simulink model "AFC2_F_trainscg_15_15_15_15_controller_ep_500_Nor_20250717"  (R2021a)
settings: Solver=VariableStepAuto  StartTime=0.0  StopTime=10.0  RelTol=1e-3
libraries: neural x66
(part 2 of 3)

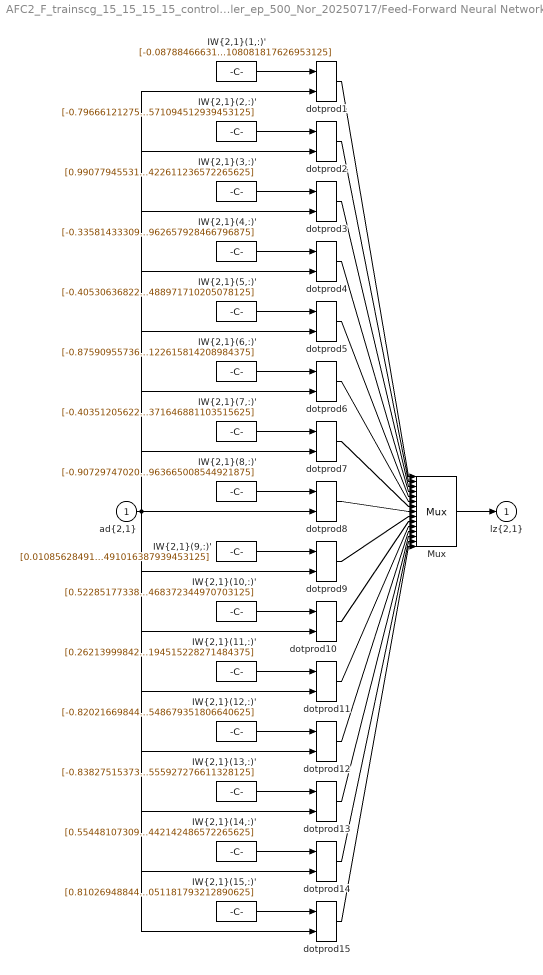
== system AFC2_F_trainscg_15_15_15_15_controller_ep_500_Nor_20250717/Feed-Forward Neural Network/Layer 2/LW{2,1} ==
  "ad{2,1}" : Inport  PortDimensions=15
      mask Display: e = 0.06;c1 = [120 230 180]/255;c2 = ([120 230 180]+0)/(256+128);c3 = ([120 230 180]+128)/(256+128);patch([0 1 1 0],[0 0 1 1],c1);patch([0 1 1 1-e 1-e 0+e],[0 0 1 1-e 0+e 0+e],c2);patch([0 0 1 1-e 0+e 0+e],[0 1 1 1-e 1-e 0+e],c3);plot([0 1 1 0 0],[0 0 1 1 0]);
  "IW{2,1}(1,:)'" : Constant  Value=[-0.0878846663125170124430951545946300029754638671875;0.06775174892635017764863647471429430879652500152587890625;0.385060464315723993689033477494376711547374725341796875;-0.8973191118577101832443077000789344310760498046875;0.4800646559755552544856982422061264514923095703125;-0.60641376213614639478777235126472078263759613037109375;-0.7754320756879466980393544872640632092952728271484375;-0.03645452907563362376919258167617954313755035400390625;-0.81526323382648147042317532395827583968639373779296875;-0.367884988017231240320370488916523754596710205078125;0.97615990087424953092209989335970021784305572509765625;-0.31661933240200113015561100837658159434795379638671875;-0.7502406969507842138256137332064099609851837158203125;-0.07347884281256167327001094236038625240325927734375;0.61840770258758670507859278586693108081817626953125]
      mask Display: e = 0.06;c1 = [120 150 230]/255;c2 = ([120 150 230]+0)/383;c3 = ([120 150 230]+128)/383;patch([0 1 1 0],[0 0 1 1],c1);patch([0 1 1 1-e 1-e 0+e],[0 0 1 1-e 0+e 0+e],c2);patch([0 0 1 1-e 0+e 0+e],[0 1 1 1-e 1-e 0+e],c3);plot([0 1 1 0 0],[0 0 1 1 0]);disp('weights');
  "IW{2,1}(10,:)'" : Constant  Value=[0.5228517733802267031251176376827061176300048828125;0.20693596766153898869333715992979705333709716796875;-0.7442232404340096696415685073588974773883819580078125;-0.7650142956963341678289225455955602228641510009765625;0.1958832707677782281052714097313582897186279296875;-0.4115421196069359854874392112833447754383087158203125;0.3109960796070747601760331235709600150585174560546875;-0.88112125053411405328773753353743813931941986083984375;-0.731393391372850754095225056516937911510467529296875;0.82788407804859354133242277384852059185504913330078125;0.2413438943991568219615828638779930770397186279296875;-0.154255850726072007983447065271320752799510955810546875;0.5277958885729565619016057098633609712123870849609375;0.4054046139009506166672736071632243692874908447265625;-0.489226519023898465121646950137801468372344970703125]
      mask Display: e = 0.06;c1 = [120 150 230]/255;c2 = ([120 150 230]+0)/383;c3 = ([120 150 230]+128)/383;patch([0 1 1 0],[0 0 1 1],c1);patch([0 1 1 1-e 1-e 0+e],[0 0 1 1-e 0+e 0+e],c2);patch([0 0 1 1-e 0+e 0+e],[0 1 1 1-e 1-e 0+e],c3);plot([0 1 1 0 0],[0 0 1 1 0]);disp('weights');
  "IW{2,1}(11,:)'" : Constant  Value=[0.262139998427187048690711890230886638164520263671875;0.0522049315911223832387122456566430628299713134765625;0.0990802140303959077982653980143368244171142578125;0.2814358459318511140878626974881626665592193603515625;0.5787278872838108600973328066174872219562530517578125;-0.5252539605888415508161415345966815948486328125;-0.780489898553896832567033925442956387996673583984375;-0.3683771233222679075680616733734495937824249267578125;-0.8028118145780045455950357791152782738208770751953125;0.4134304353938611509278189259930513799190521240234375;-0.691260389041455258762880475842393934726715087890625;-0.2807873640555287320097477277158759534358978271484375;0.518654766262192534753694417304359376430511474609375;-0.692819246761199547535170495393685996532440185546875;-0.9589284506836308619170949896215461194515228271484375]
      mask Display: e = 0.06;c1 = [120 150 230]/255;c2 = ([120 150 230]+0)/383;c3 = ([120 150 230]+128)/383;patch([0 1 1 0],[0 0 1 1],c1);patch([0 1 1 1-e 1-e 0+e],[0 0 1 1-e 0+e 0+e],c2);patch([0 0 1 1-e 0+e 0+e],[0 1 1 1-e 1-e 0+e],c3);plot([0 1 1 0 0],[0 0 1 1 0]);disp('weights');
  "IW{2,1}(12,:)'" : Constant  Value=[-0.8202166984478165279170980284106917679309844970703125;0.2472596760229174017720055189784034155309200286865234375;-0.03130315437321791460778541704712552018463611602783203125;-0.25779005620817307953274166720802895724773406982421875;-0.26469416312424609571962719201110303401947021484375;0.273188766533149329784890824157628230750560760498046875;0.86751969677066487207639511325396597385406494140625;0.6303759335450056511263028369285166263580322265625;-0.69044021123110133064670890234992839395999908447265625;-0.023850347134512041302745188886547111906111240386962890625;-0.211816580907498830388391297674388624727725982666015625;0.06174872535074608925764749756126548163592815399169921875;0.481829751237097259064512400072999298572540283203125;0.90691413977249535349756115465424954891204833984375;0.8473512252408144096449404969462193548679351806640625]
      mask Display: e = 0.06;c1 = [120 150 230]/255;c2 = ([120 150 230]+0)/383;c3 = ([120 150 230]+128)/383;patch([0 1 1 0],[0 0 1 1],c1);patch([0 1 1 1-e 1-e 0+e],[0 0 1 1-e 0+e 0+e],c2);patch([0 0 1 1-e 0+e 0+e],[0 1 1 1-e 1-e 0+e],c3);plot([0 1 1 0 0],[0 0 1 1 0]);disp('weights');
  "IW{2,1}(13,:)'" : Constant  Value=[-0.8382751537393726692926065879873931407928466796875;0.414506970630843074587801311281509697437286376953125;0.7809513583688765248069785229745320975780487060546875;0.3076240451915472906563309152261354029178619384765625;-0.5879442809896107124956188272335566580295562744140625;-0.82060262315297738400232674393919296562671661376953125;-0.62507838715662700224129366688430309295654296875;0.38755084301493669673988051727064885199069976806640625;-0.6634974030169444869642347839544527232646942138671875;-0.374899537179466724179377479231334291398525238037109375;-0.6777314823067481786011967415106482803821563720703125;0.47876521781964653801111353459418751299381256103515625;0.4873766829746519757549094720161519944667816162109375;0.0817681624829529329900879019987769424915313720703125;0.3073997780165058646417719501187093555927276611328125]
      mask Display: e = 0.06;c1 = [120 150 230]/255;c2 = ([120 150 230]+0)/383;c3 = ([120 150 230]+128)/383;patch([0 1 1 0],[0 0 1 1],c1);patch([0 1 1 1-e 1-e 0+e],[0 0 1 1-e 0+e 0+e],c2);patch([0 0 1 1-e 0+e 0+e],[0 1 1 1-e 1-e 0+e],c3);plot([0 1 1 0 0],[0 0 1 1 0]);disp('weights');
  "IW{2,1}(14,:)'" : Constant  Value=[0.554481073097886412170964831602759659290313720703125;0.5627541035985543782516060673515312373638153076171875;0.597920557625758686270955877262167632579803466796875;0.498262926207038159276407895958982408046722412109375;-0.8266669052089354874368609671364538371562957763671875;-0.189369160238817446639814079389907419681549072265625;-0.4676423221847223476999033664469607174396514892578125;-0.7493356377816400293312426583725027740001678466796875;-0.6075021554860893235883168017608113586902618408203125;-0.6675928741956986822714270601863972842693328857421875;0.516224862654837135522711832891218364238739013671875;-0.1513304327486186817708357921219430863857269287109375;-0.7881591665344693797834452198003418743610382080078125;0.3594677964209338494327994339982978999614715576171875;0.8652271440971281979415152818546630442142486572265625]
      mask Display: e = 0.06;c1 = [120 150 230]/255;c2 = ([120 150 230]+0)/383;c3 = ([120 150 230]+128)/383;patch([0 1 1 0],[0 0 1 1],c1);patch([0 1 1 1-e 1-e 0+e],[0 0 1 1-e 0+e 0+e],c2);patch([0 0 1 1-e 0+e 0+e],[0 1 1 1-e 1-e 0+e],c3);plot([0 1 1 0 0],[0 0 1 1 0]);disp('weights');
  "IW{2,1}(15,:)'" : Constant  Value=[0.810269488447141750242508351220749318599700927734375;-0.424046048771657524412148632109165191650390625;0.4686821673919394637408686321577988564968109130859375;0.1663714629097523545198100691777653992176055908203125;0.543867834198214605834209578461013734340667724609375;-0.790307304190327020165796056971885263919830322265625;0.5956605204231941730341759466682560741901397705078125;-0.7396970992211528983517609958653338253498077392578125;-0.36504044970112925483363142120651900768280029296875;0.244994582064439025970159491407684981822967529296875;0.7422222438307783942690321055124513804912567138671875;-0.1412881308849082417911091624773689545691013336181640625;0.3631208609406313403411559193045832216739654541015625;-0.926873963903094288951933776843361556529998779296875;-0.6729752629449488043889004984521307051181793212890625]
      mask Display: e = 0.06;c1 = [120 150 230]/255;c2 = ([120 150 230]+0)/383;c3 = ([120 150 230]+128)/383;patch([0 1 1 0],[0 0 1 1],c1);patch([0 1 1 1-e 1-e 0+e],[0 0 1 1-e 0+e 0+e],c2);patch([0 0 1 1-e 0+e 0+e],[0 1 1 1-e 1-e 0+e],c3);plot([0 1 1 0 0],[0 0 1 1 0]);disp('weights');
  "IW{2,1}(2,:)'" : Constant  Value=[-0.7966612127504897333807321047061122953891754150390625;-1.0766944439080428086441543200635351240634918212890625;0.1082001892355971273129711107685579918324947357177734375;-0.7153346012591350611131701953127048909664154052734375;-0.530346170504191416483763532596640288829803466796875;-0.112530674013214093687196282189688645303249359130859375;0.5688557814878254514923128226655535399913787841796875;0.65169344071455370670520323983510024845600128173828125;-0.9528829808403223022850170309538953006267547607421875;-0.498930486024516006704487836032058112323284149169921875;-0.64958838734927548674846775611513294279575347900390625;0.35345638821586522482220971141941845417022705078125;-0.94870227449216282256116983262472786009311676025390625;-0.5756735894901312544646998503594659268856048583984375;0.4972377435523942512674011595663614571094512939453125]
      mask Display: e = 0.06;c1 = [120 150 230]/255;c2 = ([120 150 230]+0)/383;c3 = ([120 150 230]+128)/383;patch([0 1 1 0],[0 0 1 1],c1);patch([0 1 1 1-e 1-e 0+e],[0 0 1 1-e 0+e 0+e],c2);patch([0 0 1 1-e 0+e 0+e],[0 1 1 1-e 1-e 0+e],c3);plot([0 1 1 0 0],[0 0 1 1 0]);disp('weights');
  "IW{2,1}(3,:)'" : Constant  Value=[0.9907794553101834100772293822956271469593048095703125;0.64699276355253754200447247058036737143993377685546875;-0.20695841483681487460444259340874850749969482421875;-0.82294508093848228735822658563847653567790985107421875;0.4699150833921044156937796287820674479007720947265625;0.06427580211802334797521751852400484494864940643310546875;-0.416859364186138225960576164652593433856964111328125;-0.2080844447464574031858575153819401748478412628173828125;-0.15378122955226392054584039215114898979663848876953125;-0.497960891694102125715204465450369752943515777587890625;-0.4844154988559739027920159060158766806125640869140625;-0.438200669103228801493088440111023373901844024658203125;-0.419629630291659949659077710748533718287944793701171875;-0.8029625246237832580931126358336769044399261474609375;-0.7596259640258387069167156369076110422611236572265625]
      mask Display: e = 0.06;c1 = [120 150 230]/255;c2 = ([120 150 230]+0)/383;c3 = ([120 150 230]+128)/383;patch([0 1 1 0],[0 0 1 1],c1);patch([0 1 1 1-e 1-e 0+e],[0 0 1 1-e 0+e 0+e],c2);patch([0 0 1 1-e 0+e 0+e],[0 1 1 1-e 1-e 0+e],c3);plot([0 1 1 0 0],[0 0 1 1 0]);disp('weights');
  "IW{2,1}(4,:)'" : Constant  Value=[-0.335814333095001860129968918045051395893096923828125;-0.3238045623956562479861531755886971950531005859375;-0.8768186658920706921804821831756271421909332275390625;0.5967017282279047929449689036118797957897186279296875;0.94119705017322896622999905957840383052825927734375;-0.54119677378130448541782016036449931561946868896484375;0.207066877501773660696926526725292205810546875;-0.453886991560920105559517878646147437393665313720703125;0.3111463498758286760903501999564468860626220703125;0.786704430823791600602135076769627630710601806640625;-0.2064013627337126788319210390909574925899505615234375;0.06251065725207975709576402323364163748919963836669921875;-0.3649588342015472886004090469214133918285369873046875;0.64714894785567711466001128428615629673004150390625;0.0500903295252175251306425707298330962657928466796875]
      mask Display: e = 0.06;c1 = [120 150 230]/255;c2 = ([120 150 230]+0)/383;c3 = ([120 150 230]+128)/383;patch([0 1 1 0],[0 0 1 1],c1);patch([0 1 1 1-e 1-e 0+e],[0 0 1 1-e 0+e 0+e],c2);patch([0 0 1 1-e 0+e 0+e],[0 1 1 1-e 1-e 0+e],c3);plot([0 1 1 0 0],[0 0 1 1 0]);disp('weights');
  "IW{2,1}(5,:)'" : Constant  Value=[-0.4053063682241566656472286922507919371128082275390625;-0.49362205125651847925638548986171372234821319580078125;0.55741736675557296276650731670088134706020355224609375;1.039281611915721104111298700445331633090972900390625;0.7338605835038318758734021685086190700531005859375;0.54500674005884264250454407374490983784198760986328125;0.928845334431802616137474615243263542652130126953125;-0.81474133701129758389214430280844680964946746826171875;0.49718119798603055414787377230823040008544921875;0.300057556973001016142887920068460516631603240966796875;-0.858379921715620497479903860948979854583740234375;0.55338634670979158780568241127184592187404632568359375;0.3070098206430660336963001100230030715465545654296875;-0.64998052523584082251772997551597654819488525390625;-0.3483327424735016553114519410883076488971710205078125]
      mask Display: e = 0.06;c1 = [120 150 230]/255;c2 = ([120 150 230]+0)/383;c3 = ([120 150 230]+128)/383;patch([0 1 1 0],[0 0 1 1],c1);patch([0 1 1 1-e 1-e 0+e],[0 0 1 1-e 0+e 0+e],c2);patch([0 0 1 1-e 0+e 0+e],[0 1 1 1-e 1-e 0+e],c3);plot([0 1 1 0 0],[0 0 1 1 0]);disp('weights');
  "IW{2,1}(6,:)'" : Constant  Value=[-0.8759095573607347251510191199486143887042999267578125;0.71296833252932412250402194331400096416473388671875;-0.32055590564301750244879940510145388543605804443359375;0.256503357960496780609815914431237615644931793212890625;-0.8275309402730073315979097969830036163330078125;-0.264412403108604754375932088805711828172206878662109375;-0.135030012059278003988538330304436385631561279296875;0.15100948477099895850273014730191789567470550537109375;0.04367294366911933511943288976908661425113677978515625;-0.0301408993288969605239824289810712798498570919036865234375;0.356621360229519179796398020698688924312591552734375;0.1145468995769869102741012056867475621402263641357421875;0.91469259624341514580692091840319335460662841796875;-0.672860180430013610219930342282168567180633544921875;0.0928988798061369802638864712207578122615814208984375]
      mask Display: e = 0.06;c1 = [120 150 230]/255;c2 = ([120 150 230]+0)/383;c3 = ([120 150 230]+128)/383;patch([0 1 1 0],[0 0 1 1],c1);patch([0 1 1 1-e 1-e 0+e],[0 0 1 1-e 0+e 0+e],c2);patch([0 0 1 1-e 0+e 0+e],[0 1 1 1-e 1-e 0+e],c3);plot([0 1 1 0 0],[0 0 1 1 0]);disp('weights');
  "IW{2,1}(7,:)'" : Constant  Value=[-0.40351205622447228194005219847895205020904541015625;-0.979326763313207226957501916331239044666290283203125;0.215731814525891518741218533250503242015838623046875;-0.735834088572874467359952177503146231174468994140625;-0.2671267673616022353400012434576638042926788330078125;-0.6963089497674668226778749158256687223911285400390625;0.3895043892358802661846084447461180388927459716796875;-0.14087108149629390396739836432971060276031494140625;-0.782364123453909154903840317274443805217742919921875;-0.631132664484693517437108312151394784450531005859375;-0.19522333460767615775921512977220118045806884765625;-0.3293773385895077954188536750734783709049224853515625;0.8714617455697608594533676296123303472995758056640625;0.3319744328222211660062157534412108361721038818359375;-0.20223849523360204472055556834675371646881103515625]
      mask Display: e = 0.06;c1 = [120 150 230]/255;c2 = ([120 150 230]+0)/383;c3 = ([120 150 230]+128)/383;patch([0 1 1 0],[0 0 1 1],c1);patch([0 1 1 1-e 1-e 0+e],[0 0 1 1-e 0+e 0+e],c2);patch([0 0 1 1-e 0+e 0+e],[0 1 1 1-e 1-e 0+e],c3);plot([0 1 1 0 0],[0 0 1 1 0]);disp('weights');
  "IW{2,1}(8,:)'" : Constant  Value=[-0.90729747020363848974966458627022802829742431640625;-0.903105321493555823764154411037452518939971923828125;0.4825080990044359197099765879102051258087158203125;0.4454490793135317261430827784352004528045654296875;-0.2616023913399636580123797102714888751506805419921875;0.5638639331760038064800255597219802439212799072265625;0.5161985505789081773997395430342294275760650634765625;-0.096521530190528892489965073764324188232421875;0.26353274705697771196355461142957210540771484375;-0.5759383149353585196195126627571880817413330078125;0.9656704027879019491820145049132406711578369140625;-0.401549953333786735498733833082951605319976806640625;-0.084227332291266332475743183749727904796600341796875;0.7887787507084855764816211376455612480640411376953125;-0.16981322677390675579545131768099963665008544921875]
      mask Display: e = 0.06;c1 = [120 150 230]/255;c2 = ([120 150 230]+0)/383;c3 = ([120 150 230]+128)/383;patch([0 1 1 0],[0 0 1 1],c1);patch([0 1 1 1-e 1-e 0+e],[0 0 1 1-e 0+e 0+e],c2);patch([0 0 1 1-e 0+e 0+e],[0 1 1 1-e 1-e 0+e],c3);plot([0 1 1 0 0],[0 0 1 1 0]);disp('weights');
  "IW{2,1}(9,:)'" : Constant  Value=[0.010856284915405911561947505106218159198760986328125;0.335832243112431039211429606439196504652500152587890625;-0.7903735160530007686219278184580616652965545654296875;-0.7792930387153027549373973670299164950847625732421875;0.3700569453232185335167514494969509541988372802734375;-0.8134134635911294264332127568195573985576629638671875;-0.1347153477057989601206600127625279128551483154296875;0.2056321119793460272529017629494774155318737030029296875;-0.7470002693413941852185189418378286063671112060546875;-0.84647755856120754369698033769964240491390228271484375;-0.195632029555030673151350129046477377414703369140625;-0.1106543357761184953602651148685254156589508056640625;-0.5190455904370330220132245813147164881229400634765625;0.0331164167025408406885844669886864721775054931640625;-0.63852447949041124530822344240732491016387939453125]
      mask Display: e = 0.06;c1 = [120 150 230]/255;c2 = ([120 150 230]+0)/383;c3 = ([120 150 230]+128)/383;patch([0 1 1 0],[0 0 1 1],c1);patch([0 1 1 1-e 1-e 0+e],[0 0 1 1-e 0+e 0+e],c2);patch([0 0 1 1-e 0+e 0+e],[0 1 1 1-e 1-e 0+e],c3);plot([0 1 1 0 0],[0 0 1 1 0]);disp('weights');
  Mux : Mux  Inputs=15
      mask Display: e = 0.06;c1 = [120 150 230]/255;c2 = ([120 150 230]+0)/383;c3 = ([120 150 230]+128)/383;patch([0 1 1 0],[0 0 1 1],c1);patch([0 1 1 1-e 1-e 0+e],[0 0 1 1-e 0+e 0+e],c2);patch([0 0 1 1-e 0+e 0+e],[0 1 1 1-e 1-e 0+e],c3);plot([0 1 1 0 0],[0 0 1 1 0]);disp('Mux');
  dotprod{1..15} (15 alike) : neural/Weight Functions/dotprod
  "lz{2,1}" : Outport
      mask Display: e = 0.06;c1 = [120 230 180]/255;c2 = ([120 230 180]+0)/(256+128);c3 = ([120 230 180]+128)/(256+128);patch([0 1 1 0],[0 0 1 1],c1);patch([0 1 1 1-e 1-e 0+e],[0 0 1 1-e 0+e 0+e],c2);patch([0 0 1 1-e 0+e 0+e],[0 1 1 1-e 1-e 0+e],c3);plot([0 1 1 0 0],[0 0 1 1 0]);
  wires:
  "IW{2,1}(1,:)'"/1 -> dotprod1/1
  "ad{2,1}"/1 -> dotprod1/2, dotprod2/2, dotprod3/2, dotprod4/2, dotprod5/2, dotprod6/2, dotprod7/2, dotprod8/2, dotprod9/2, dotprod10/2, dotprod11/2, dotprod12/2, dotprod13/2, dotprod14/2, dotprod15/2
  dotprod1/1 -> Mux/1
  "IW{2,1}(2,:)'"/1 -> dotprod2/1
  dotprod2/1 -> Mux/2
  "IW{2,1}(3,:)'"/1 -> dotprod3/1
  dotprod3/1 -> Mux/3
  "IW{2,1}(4,:)'"/1 -> dotprod4/1
  dotprod4/1 -> Mux/4
  "IW{2,1}(5,:)'"/1 -> dotprod5/1
  dotprod5/1 -> Mux/5
  "IW{2,1}(6,:)'"/1 -> dotprod6/1
  dotprod6/1 -> Mux/6
  "IW{2,1}(7,:)'"/1 -> dotprod7/1
  dotprod7/1 -> Mux/7
  "IW{2,1}(8,:)'"/1 -> dotprod8/1
  dotprod8/1 -> Mux/8
  "IW{2,1}(9,:)'"/1 -> dotprod9/1
  dotprod9/1 -> Mux/9
  "IW{2,1}(10,:)'"/1 -> dotprod10/1
  dotprod10/1 -> Mux/10
  "IW{2,1}(11,:)'"/1 -> dotprod11/1
  dotprod11/1 -> Mux/11
  "IW{2,1}(12,:)'"/1 -> dotprod12/1
  dotprod12/1 -> Mux/12
  "IW{2,1}(13,:)'"/1 -> dotprod13/1
  dotprod13/1 -> Mux/13
  "IW{2,1}(14,:)'"/1 -> dotprod14/1
  dotprod14/1 -> Mux/14
  "IW{2,1}(15,:)'"/1 -> dotprod15/1
  dotprod15/1 -> Mux/15
  Mux/1 -> "lz{2,1}"/1

== system AFC2_F_trainscg_15_15_15_15_controller_ep_500_Nor_20250717/Feed-Forward Neural Network/Layer 3/Delays 1 ==
  "p{3}" : Inport  PortDimensions=15
      mask Display: e = 0.06;c1 = [120 230 180]/255;c2 = ([120 230 180]+0)/(256+128);c3 = ([120 230 180]+128)/(256+128);patch([0 1 1 0],[0 0 1 1],c1);patch([0 1 1 1-e 1-e 0+e],[0 0 1 1-e 0+e 0+e],c2);patch([0 0 1 1-e 0+e 0+e],[0 1 1 1-e 1-e 0+e],c3);plot([0 1 1 0 0],[0 0 1 1 0]);
  mux : Mux  Inputs=1
      mask Display: e = 0.06;c1 = [120 150 230]/255;c2 = ([120 150 230]+0)/383;c3 = ([120 150 230]+128)/383;patch([0 1 1 0],[0 0 1 1],c1);patch([0 1 1 1-e 1-e 0+e],[0 0 1 1-e 0+e 0+e],c2);patch([0 0 1 1-e 0+e 0+e],[0 1 1 1-e 1-e 0+e],c3);plot([0 1 1 0 0],[0 0 1 1 0]);disp('Mux')
  "pd{3,2}" : Outport
      mask Display: e = 0.06;c1 = [120 230 180]/255;c2 = ([120 230 180]+0)/(256+128);c3 = ([120 230 180]+128)/(256+128);patch([0 1 1 0],[0 0 1 1],c1);patch([0 1 1 1-e 1-e 0+e],[0 0 1 1-e 0+e 0+e],c2);patch([0 0 1 1-e 0+e 0+e],[0 1 1 1-e 1-e 0+e],c3);plot([0 1 1 0 0],[0 0 1 1 0]);
  wires:
  "p{3}"/1 -> mux/1
  mux/1 -> "pd{3,2}"/1

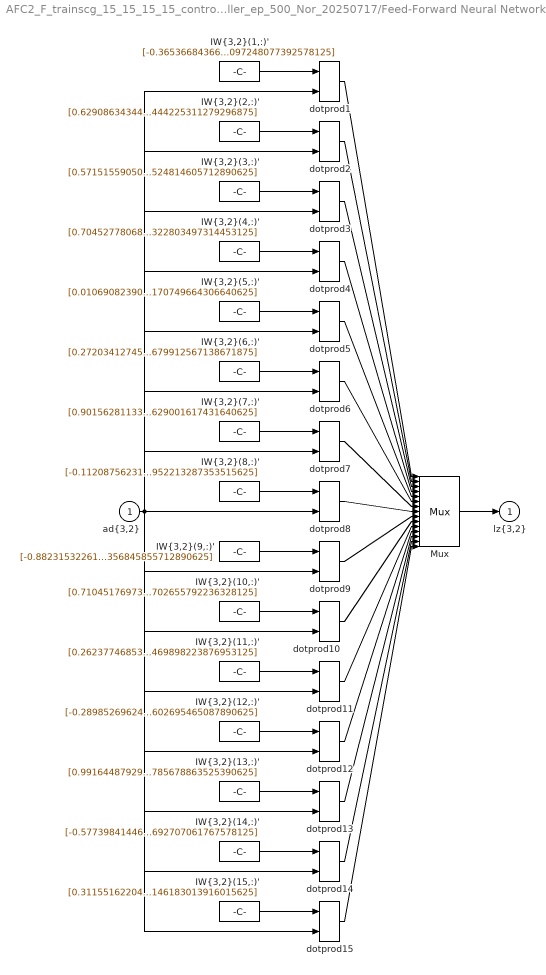
== system AFC2_F_trainscg_15_15_15_15_controller_ep_500_Nor_20250717/Feed-Forward Neural Network/Layer 3/LW{3,2} ==
  "ad{3,2}" : Inport  PortDimensions=15
      mask Display: e = 0.06;c1 = [120 230 180]/255;c2 = ([120 230 180]+0)/(256+128);c3 = ([120 230 180]+128)/(256+128);patch([0 1 1 0],[0 0 1 1],c1);patch([0 1 1 1-e 1-e 0+e],[0 0 1 1-e 0+e 0+e],c2);patch([0 0 1 1-e 0+e 0+e],[0 1 1 1-e 1-e 0+e],c3);plot([0 1 1 0 0],[0 0 1 1 0]);
  "IW{3,2}(1,:)'" : Constant  Value=[-0.365366843662218776511707574172760359942913055419921875;0.297626033948104551374314041822799481451511383056640625;-0.552576538834370634134529609582386910915374755859375;0.6262391833095402038367183195077814161777496337890625;0.994869663054350983344420455978251993656158447265625;0.2158818539358546562123564171997713856399059295654296875;-0.17681297318493083281509825610555708408355712890625;-0.17314542195836946092413199949078261852264404296875;-0.5514458586709711784834553327527828514575958251953125;0.7919867652746674924202352485735900700092315673828125;0.002565826406430549155857079313136637210845947265625;0.45504092350284419676853531200322322547435760498046875;-0.01531190268565920005461311603767171618528664112091064453125;0.32087593262520375247959236730821430683135986328125;0.0075615715317442662446456580482845311053097248077392578125]
      mask Display: e = 0.06;c1 = [120 150 230]/255;c2 = ([120 150 230]+0)/383;c3 = ([120 150 230]+128)/383;patch([0 1 1 0],[0 0 1 1],c1);patch([0 1 1 1-e 1-e 0+e],[0 0 1 1-e 0+e 0+e],c2);patch([0 0 1 1-e 0+e 0+e],[0 1 1 1-e 1-e 0+e],c3);plot([0 1 1 0 0],[0 0 1 1 0]);disp('weights');
  "IW{3,2}(10,:)'" : Constant  Value=[0.71045176973429502442769489789498038589954376220703125;0.69489864071527829292307387731852941215038299560546875;-0.2329333480080961471525569095319951884448528289794921875;0.60895706649294023549146004370413720607757568359375;0.42131106666719808639953726014937274158000946044921875;-0.4606067387734202878135647551971487700939178466796875;0.9923122225937388574124042861512862145900726318359375;0.8446639955925514531287490171962417662143707275390625;0.86756609046020838338364455921691842377185821533203125;0.0212516981011370877097110820841407985426485538482666015625;0.8349876648322338557051125462749041616916656494140625;0.0449366863013828943262950588177773170173168182373046875;0.325018768624063258965151135271298699080944061279296875;-0.7244742149609673109722507433616556227207183837890625;0.3342406008340959022717697735060937702655792236328125]
      mask Display: e = 0.06;c1 = [120 150 230]/255;c2 = ([120 150 230]+0)/383;c3 = ([120 150 230]+128)/383;patch([0 1 1 0],[0 0 1 1],c1);patch([0 1 1 1-e 1-e 0+e],[0 0 1 1-e 0+e 0+e],c2);patch([0 0 1 1-e 0+e 0+e],[0 1 1 1-e 1-e 0+e],c3);plot([0 1 1 0 0],[0 0 1 1 0]);disp('weights');
  "IW{3,2}(11,:)'" : Constant  Value=[0.26237746853802246249642848852090537548065185546875;0.142051745648757776763204674352891743183135986328125;0.25469300488693402684248212608508765697479248046875;0.9722084837919402477979247123585082590579986572265625;-0.724262015174883533319416528684087097644805908203125;0.3247637207989624297255204510292969644069671630859375;-0.290931390086156316243659603060223162174224853515625;0.5419084413478489903326362764346413314342498779296875;-0.7842221898312728978197583273868076503276824951171875;0.812728646530429532646166990161873400211334228515625;0.4271480231886315426237388237495906651020050048828125;-0.3391527807867944499520262979785911738872528076171875;-0.4369968817030187580030542449094355106353759765625;0.6734455634994349626509801964857615530490875244140625;0.172879229357835839664403465576469898223876953125]
      mask Display: e = 0.06;c1 = [120 150 230]/255;c2 = ([120 150 230]+0)/383;c3 = ([120 150 230]+128)/383;patch([0 1 1 0],[0 0 1 1],c1);patch([0 1 1 1-e 1-e 0+e],[0 0 1 1-e 0+e 0+e],c2);patch([0 0 1 1-e 0+e 0+e],[0 1 1 1-e 1-e 0+e],c3);plot([0 1 1 0 0],[0 0 1 1 0]);disp('weights');
  "IW{3,2}(12,:)'" : Constant  Value=[-0.2898526962423020325587685874779708683490753173828125;-0.646289884749394527574395397095941007137298583984375;-0.9567003707393870737263341652578674256801605224609375;-0.940016099461220111521697617718018591403961181640625;-0.5643968125757508058626399360946379601955413818359375;-0.511669426419441464304327382706105709075927734375;0.9425176303668114652367648886865936219692230224609375;-0.9146802881299025411721004275023005902767181396484375;-0.6355449887978885659123307050322182476520538330078125;0.2578478773046357641618442357867024838924407958984375;0.2366747672438800353944543530815280973911285400390625;0.238943110355559706903250116738490760326385498046875;-0.5392338653650725621702122225542552769184112548828125;-0.7227965685152799579782367800362408161163330078125;0.3502248328102306462739079506718553602695465087890625]
      mask Display: e = 0.06;c1 = [120 150 230]/255;c2 = ([120 150 230]+0)/383;c3 = ([120 150 230]+128)/383;patch([0 1 1 0],[0 0 1 1],c1);patch([0 1 1 1-e 1-e 0+e],[0 0 1 1-e 0+e 0+e],c2);patch([0 0 1 1-e 0+e 0+e],[0 1 1 1-e 1-e 0+e],c3);plot([0 1 1 0 0],[0 0 1 1 0]);disp('weights');
  "IW{3,2}(13,:)'" : Constant  Value=[0.991644879297117309846498756087385118007659912109375;0.90108329341554116442836175338015891611576080322265625;0.82113984593669775424729095902875997126102447509765625;0.07132838133447538808695753687061369419097900390625;-0.6357747147812780053044434680487029254436492919921875;-0.41455579669982489665613911711261607706546783447265625;-0.3071024773992807599398702222970314323902130126953125;-0.243627725899562275202470118529163300991058349609375;-0.80207359330083594084470632878947071731090545654296875;-0.7969322223753756428976657844032160937786102294921875;-0.313424219517309143867578313802368938922882080078125;-0.2873017552382091110985129489563405513763427734375;0.422208944759932591761497633342514745891094207763671875;0.17641877077898726611238089390099048614501953125;-0.2779559016106782909361072597675956785678863525390625]
      mask Display: e = 0.06;c1 = [120 150 230]/255;c2 = ([120 150 230]+0)/383;c3 = ([120 150 230]+128)/383;patch([0 1 1 0],[0 0 1 1],c1);patch([0 1 1 1-e 1-e 0+e],[0 0 1 1-e 0+e 0+e],c2);patch([0 0 1 1-e 0+e 0+e],[0 1 1 1-e 1-e 0+e],c3);plot([0 1 1 0 0],[0 0 1 1 0]);disp('weights');
  "IW{3,2}(14,:)'" : Constant  Value=[-0.57739841446789841317155378419556654989719390869140625;-0.30550652972354475078731184112257324159145355224609375;0.59942099184168318171117562087601982057094573974609375;-0.82583098587346182029023111681453883647918701171875;-0.87729538964294617731098924195975996553897857666015625;0.1779466910312280381045724197974777780473232269287109375;0.7730877235206126130151460529305040836334228515625;0.4086792489667352423765578350867144763469696044921875;-0.021993297039783345214747356521911569871008396148681640625;-0.2180143728547492276703678726335056126117706298828125;0.8720546533795394683608037666999734938144683837890625;0.42705524927352678243863692841841839253902435302734375;0.24885189656073791741874856597860343754291534423828125;-0.267686399090124371724641605396755039691925048828125;0.2405568552264379100780189446595613844692707061767578125]
      mask Display: e = 0.06;c1 = [120 150 230]/255;c2 = ([120 150 230]+0)/383;c3 = ([120 150 230]+128)/383;patch([0 1 1 0],[0 0 1 1],c1);patch([0 1 1 1-e 1-e 0+e],[0 0 1 1-e 0+e 0+e],c2);patch([0 0 1 1-e 0+e 0+e],[0 1 1 1-e 1-e 0+e],c3);plot([0 1 1 0 0],[0 0 1 1 0]);disp('weights');
  "IW{3,2}(15,:)'" : Constant  Value=[0.311551622049496879096608381587429903447628021240234375;0.90390423524640273189589834146318025887012481689453125;0.491695034966646515872668032898218370974063873291015625;0.604182881111607894553117148461751639842987060546875;-0.7844616745964099191468221761169843375682830810546875;0.06569214114054984510193690994128701277077198028564453125;-0.09061027001618437992647159262560307979583740234375;0.4590260910092938129167805527686141431331634521484375;-0.612990217470481102424173514009453356266021728515625;-0.89076676955268485613714801729656755924224853515625;-0.7504519186790148399524014166672714054584503173828125;-0.159467956548511369252452141154208220541477203369140625;0.181316781990532749357925013100611977279186248779296875;0.6135190893222113306393339371425099670886993408203125;0.6223017702005704254730744651169516146183013916015625]
      mask Display: e = 0.06;c1 = [120 150 230]/255;c2 = ([120 150 230]+0)/383;c3 = ([120 150 230]+128)/383;patch([0 1 1 0],[0 0 1 1],c1);patch([0 1 1 1-e 1-e 0+e],[0 0 1 1-e 0+e 0+e],c2);patch([0 0 1 1-e 0+e 0+e],[0 1 1 1-e 1-e 0+e],c3);plot([0 1 1 0 0],[0 0 1 1 0]);disp('weights');
  "IW{3,2}(2,:)'" : Constant  Value=[0.62908634344232883250924714957363903522491455078125;-0.2464814889793518204452738018517266027629375457763671875;-0.252872384643419823024856896154233254492282867431640625;-0.23338736274894156252912580384872853755950927734375;-0.86512205740391812103240454234764911234378814697265625;0.8962787457970764481984815574833191931247711181640625;0.20527643607279433268786306143738329410552978515625;-0.5645358632853991753819400400971062481403350830078125;-0.46189044751869168248248342933948151767253875732421875;-0.801820700636370897740334839909337460994720458984375;-0.1365576562315056197149942818214185535907745361328125;0.277707499761643716862380415477673523128032684326171875;0.389486467026595672979993878470850177109241485595703125;-0.904890653772267850030175395659171044826507568359375;-0.0208113225532915446791548674809746444225311279296875]
      mask Display: e = 0.06;c1 = [120 150 230]/255;c2 = ([120 150 230]+0)/383;c3 = ([120 150 230]+128)/383;patch([0 1 1 0],[0 0 1 1],c1);patch([0 1 1 1-e 1-e 0+e],[0 0 1 1-e 0+e 0+e],c2);patch([0 0 1 1-e 0+e 0+e],[0 1 1 1-e 1-e 0+e],c3);plot([0 1 1 0 0],[0 0 1 1 0]);disp('weights');
  "IW{3,2}(3,:)'" : Constant  Value=[0.571515590501291637082204033504240214824676513671875;-0.6200892262707096147522634055349044501781463623046875;-0.82518679669478889326938997328397817909717559814453125;0.234560136476551439610460647600120864808559417724609375;0.94283428316362438703635007186676375567913055419921875;-0.308277913399540415273492044434533454477787017822265625;0.5010401118474712145456351208849810063838958740234375;-0.748690825274747506767880622646771371364593505859375;0.34552491106998772796288221798022277653217315673828125;-0.91162696781648211441506646224297583103179931640625;0.9951206990243781635996356271789409220218658447265625;0.6813094448454537488402138478704728186130523681640625;0.9453529234626014687847828099620528519153594970703125;-0.302430382979882228511314679053612053394317626953125;0.75409744717475357678182490417384542524814605712890625]
      mask Display: e = 0.06;c1 = [120 150 230]/255;c2 = ([120 150 230]+0)/383;c3 = ([120 150 230]+128)/383;patch([0 1 1 0],[0 0 1 1],c1);patch([0 1 1 1-e 1-e 0+e],[0 0 1 1-e 0+e 0+e],c2);patch([0 0 1 1-e 0+e 0+e],[0 1 1 1-e 1-e 0+e],c3);plot([0 1 1 0 0],[0 0 1 1 0]);disp('weights');
  "IW{3,2}(4,:)'" : Constant  Value=[0.7045277806876912851663519177236594259738922119140625;-0.94973037652686420617698104251758195459842681884765625;0.28023309649343008942423693952150642871856689453125;0.1509897194056277758278383771539665758609771728515625;-0.9636452104287036579677305780933238565921783447265625;-0.17911605323829993263728965757763944566249847412109375;0.1670663485239172185714551233104430139064788818359375;-0.3821708128663694470361633648280985653400421142578125;-0.0450156045462775100673979977727867662906646728515625;0.1145903116095237095350967138074338436126708984375;0.623205161990645795100363102392293512821197509765625;-0.2035708272204545810080134060626733116805553436279296875;-0.3444900790131864010135132048162631690502166748046875;-0.0973188392885135922227846094756387174129486083984375;-0.2937163741220889523475534588214941322803497314453125]
      mask Display: e = 0.06;c1 = [120 150 230]/255;c2 = ([120 150 230]+0)/383;c3 = ([120 150 230]+128)/383;patch([0 1 1 0],[0 0 1 1],c1);patch([0 1 1 1-e 1-e 0+e],[0 0 1 1-e 0+e 0+e],c2);patch([0 0 1 1-e 0+e 0+e],[0 1 1 1-e 1-e 0+e],c3);plot([0 1 1 0 0],[0 0 1 1 0]);disp('weights');
  "IW{3,2}(5,:)'" : Constant  Value=[0.010690823907084957833379945668639265932142734527587890625;-0.1719766364448367668149586506842751987278461456298828125;-0.6390499182001569966615761586581356823444366455078125;0.06010214199132594969920972971522132866084575653076171875;0.3551902092111427489129482637508772313594818115234375;0.9431980029510584895291458451538346707820892333984375;0.1035850298719349638076892006210982799530029296875;0.4522088633296637016911745377001352608203887939453125;0.2474359349173319844172880266341962851583957672119140625;0.5449380348425252318378397831111215054988861083984375;-0.0286966602039646634381142575875855982303619384765625;0.46471794347871397956595274081337265670299530029296875;0.67559858175389486678596995261614210903644561767578125;-0.518190005759778582472563357441686093807220458984375;-0.1011128867059986335963372994228848256170749664306640625]
      mask Display: e = 0.06;c1 = [120 150 230]/255;c2 = ([120 150 230]+0)/383;c3 = ([120 150 230]+128)/383;patch([0 1 1 0],[0 0 1 1],c1);patch([0 1 1 1-e 1-e 0+e],[0 0 1 1-e 0+e 0+e],c2);patch([0 0 1 1-e 0+e 0+e],[0 1 1 1-e 1-e 0+e],c3);plot([0 1 1 0 0],[0 0 1 1 0]);disp('weights');
  "IW{3,2}(6,:)'" : Constant  Value=[0.272034127452681462333572426359751261770725250244140625;-0.737460157290359408222002457478083670139312744140625;-0.90980217796257167872653326412546448409557342529296875;-0.449900488194286352072737145135761238634586334228515625;0.494289335168418719756999735182034783065319061279296875;0.93137012662846141441974623376154340803623199462890625;0.1671412375154288643130939817638136446475982666015625;0.565744145958246402727809254429303109645843505859375;-0.5271113019032112045891835805377922952175140380859375;-0.37677324251806576516088398420833982527256011962890625;0.7888955111347863979887051755213178694248199462890625;0.7259618129295331012684755478403531014919281005859375;0.478181606638909684203753158726613037288188934326171875;0.430090026592353069645469076931476593017578125;0.92706057341037506613901086893747560679912567138671875]
      mask Display: e = 0.06;c1 = [120 150 230]/255;c2 = ([120 150 230]+0)/383;c3 = ([120 150 230]+128)/383;patch([0 1 1 0],[0 0 1 1],c1);patch([0 1 1 1-e 1-e 0+e],[0 0 1 1-e 0+e 0+e],c2);patch([0 0 1 1-e 0+e 0+e],[0 1 1 1-e 1-e 0+e],c3);plot([0 1 1 0 0],[0 0 1 1 0]);disp('weights');
  "IW{3,2}(7,:)'" : Constant  Value=[0.9015628113306479729516240695375017821788787841796875;0.45035426531354261214801226742565631866455078125;0.446346958366190538214368643821217119693756103515625;-0.5027420806760591887041300651617348194122314453125;0.06827512505080635119014687006711028516292572021484375;0.352738022646406135240937373964698053896427154541015625;0.02363983991695040032254837569780647754669189453125;0.3875752299737944550628299111849628388881683349609375;-0.64580752386085948923977184676914475858211517333984375;-0.642035041371329828763236946542747318744659423828125;-0.7249068104658704658760370875825174152851104736328125;-0.35575371679816758518910546627012081444263458251953125;0.90828996621275959189034665541839785873889923095703125;0.7123645840125758521566012859693728387355804443359375;-0.9154044041709143986196295372792519629001617431640625]
      mask Display: e = 0.06;c1 = [120 150 230]/255;c2 = ([120 150 230]+0)/383;c3 = ([120 150 230]+128)/383;patch([0 1 1 0],[0 0 1 1],c1);patch([0 1 1 1-e 1-e 0+e],[0 0 1 1-e 0+e 0+e],c2);patch([0 0 1 1-e 0+e 0+e],[0 1 1 1-e 1-e 0+e],c3);plot([0 1 1 0 0],[0 0 1 1 0]);disp('weights');
  "IW{3,2}(8,:)'" : Constant  Value=[-0.11208756231303330930249018138056271709501743316650390625;-0.255363811844343313595118161174468696117401123046875;-0.305225945888636551739381275183404795825481414794921875;-0.09671943368445302946501129781609051860868930816650390625;0.748904075602730312510857402230612933635711669921875;0.9708972453838555782823505069245584309101104736328125;-0.8348145460026012987242438612156547605991363525390625;-0.98039549547387583317004100535996258258819580078125;0.6592866677039992406861301788012497127056121826171875;-0.322046757474971301338229068278451450169086456298828125;-0.2199901711094292000581162938033230602741241455078125;0.10442364182115755621982344791831565089523792266845703125;-0.936154741609782181654964006156660616397857666015625;-0.4369846097628933279111151932738721370697021484375;0.945916668183953479598358171642757952213287353515625]
      mask Display: e = 0.06;c1 = [120 150 230]/255;c2 = ([120 150 230]+0)/383;c3 = ([120 150 230]+128)/383;patch([0 1 1 0],[0 0 1 1],c1);patch([0 1 1 1-e 1-e 0+e],[0 0 1 1-e 0+e 0+e],c2);patch([0 0 1 1-e 0+e 0+e],[0 1 1 1-e 1-e 0+e],c3);plot([0 1 1 0 0],[0 0 1 1 0]);disp('weights');
  "IW{3,2}(9,:)'" : Constant  Value=[-0.88231532261132283867510750496876426041126251220703125;0.72990198785852478113866936837439425289630889892578125;0.321080088187972345625809111879789270460605621337890625;-0.5445536507185124719399027526378631591796875;0.8452432411959909241971899973577819764614105224609375;0.48964339599453676754592379438690841197967529296875;0.4391402697189794590570954824215732514858245849609375;0.686426676021019144258161759353242814540863037109375;0.5337885882454587171963567016064189374446868896484375;-0.57938728560713081972011195830418728291988372802734375;0.854712449996249734596176494960673153400421142578125;0.90773356474495903167820642920560203492641448974609375;-0.28628441346536337430705998485791496932506561279296875;0.46210165944748293753718826337717473506927490234375;-0.62158631370082506606422612094320356845855712890625]
      mask Display: e = 0.06;c1 = [120 150 230]/255;c2 = ([120 150 230]+0)/383;c3 = ([120 150 230]+128)/383;patch([0 1 1 0],[0 0 1 1],c1);patch([0 1 1 1-e 1-e 0+e],[0 0 1 1-e 0+e 0+e],c2);patch([0 0 1 1-e 0+e 0+e],[0 1 1 1-e 1-e 0+e],c3);plot([0 1 1 0 0],[0 0 1 1 0]);disp('weights');
  Mux : Mux  Inputs=15
      mask Display: e = 0.06;c1 = [120 150 230]/255;c2 = ([120 150 230]+0)/383;c3 = ([120 150 230]+128)/383;patch([0 1 1 0],[0 0 1 1],c1);patch([0 1 1 1-e 1-e 0+e],[0 0 1 1-e 0+e 0+e],c2);patch([0 0 1 1-e 0+e 0+e],[0 1 1 1-e 1-e 0+e],c3);plot([0 1 1 0 0],[0 0 1 1 0]);disp('Mux');
  dotprod{1..15} (15 alike) : neural/Weight Functions/dotprod
  "lz{3,2}" : Outport
      mask Display: e = 0.06;c1 = [120 230 180]/255;c2 = ([120 230 180]+0)/(256+128);c3 = ([120 230 180]+128)/(256+128);patch([0 1 1 0],[0 0 1 1],c1);patch([0 1 1 1-e 1-e 0+e],[0 0 1 1-e 0+e 0+e],c2);patch([0 0 1 1-e 0+e 0+e],[0 1 1 1-e 1-e 0+e],c3);plot([0 1 1 0 0],[0 0 1 1 0]);
  wires:
  "IW{3,2}(1,:)'"/1 -> dotprod1/1
  "ad{3,2}"/1 -> dotprod1/2, dotprod2/2, dotprod3/2, dotprod4/2, dotprod5/2, dotprod6/2, dotprod7/2, dotprod8/2, dotprod9/2, dotprod10/2, dotprod11/2, dotprod12/2, dotprod13/2, dotprod14/2, dotprod15/2
  dotprod1/1 -> Mux/1
  "IW{3,2}(2,:)'"/1 -> dotprod2/1
  dotprod2/1 -> Mux/2
  "IW{3,2}(3,:)'"/1 -> dotprod3/1
  dotprod3/1 -> Mux/3
  "IW{3,2}(4,:)'"/1 -> dotprod4/1
  dotprod4/1 -> Mux/4
  "IW{3,2}(5,:)'"/1 -> dotprod5/1
  dotprod5/1 -> Mux/5
  "IW{3,2}(6,:)'"/1 -> dotprod6/1
  dotprod6/1 -> Mux/6
  "IW{3,2}(7,:)'"/1 -> dotprod7/1
  dotprod7/1 -> Mux/7
  "IW{3,2}(8,:)'"/1 -> dotprod8/1
  dotprod8/1 -> Mux/8
  "IW{3,2}(9,:)'"/1 -> dotprod9/1
  dotprod9/1 -> Mux/9
  "IW{3,2}(10,:)'"/1 -> dotprod10/1
  dotprod10/1 -> Mux/10
  "IW{3,2}(11,:)'"/1 -> dotprod11/1
  dotprod11/1 -> Mux/11
  "IW{3,2}(12,:)'"/1 -> dotprod12/1
  dotprod12/1 -> Mux/12
  "IW{3,2}(13,:)'"/1 -> dotprod13/1
  dotprod13/1 -> Mux/13
  "IW{3,2}(14,:)'"/1 -> dotprod14/1
  dotprod14/1 -> Mux/14
  "IW{3,2}(15,:)'"/1 -> dotprod15/1
  dotprod15/1 -> Mux/15
  Mux/1 -> "lz{3,2}"/1

== system AFC2_F_trainscg_15_15_15_15_controller_ep_500_Nor_20250717/Feed-Forward Neural Network/Layer 4/Delays 1 ==
  "p{4}" : Inport  PortDimensions=15
      mask Display: e = 0.06;c1 = [120 230 180]/255;c2 = ([120 230 180]+0)/(256+128);c3 = ([120 230 180]+128)/(256+128);patch([0 1 1 0],[0 0 1 1],c1);patch([0 1 1 1-e 1-e 0+e],[0 0 1 1-e 0+e 0+e],c2);patch([0 0 1 1-e 0+e 0+e],[0 1 1 1-e 1-e 0+e],c3);plot([0 1 1 0 0],[0 0 1 1 0]);
  mux : Mux  Inputs=1
      mask Display: e = 0.06;c1 = [120 150 230]/255;c2 = ([120 150 230]+0)/383;c3 = ([120 150 230]+128)/383;patch([0 1 1 0],[0 0 1 1],c1);patch([0 1 1 1-e 1-e 0+e],[0 0 1 1-e 0+e 0+e],c2);patch([0 0 1 1-e 0+e 0+e],[0 1 1 1-e 1-e 0+e],c3);plot([0 1 1 0 0],[0 0 1 1 0]);disp('Mux')
  "pd{4,3}" : Outport
      mask Display: e = 0.06;c1 = [120 230 180]/255;c2 = ([120 230 180]+0)/(256+128);c3 = ([120 230 180]+128)/(256+128);patch([0 1 1 0],[0 0 1 1],c1);patch([0 1 1 1-e 1-e 0+e],[0 0 1 1-e 0+e 0+e],c2);patch([0 0 1 1-e 0+e 0+e],[0 1 1 1-e 1-e 0+e],c3);plot([0 1 1 0 0],[0 0 1 1 0]);
  wires:
  "p{4}"/1 -> mux/1
  mux/1 -> "pd{4,3}"/1
